simulink model "P2_B"  (R2024b)
settings: Solver=VariableStepAuto  StartTime=0.0  StopTime=10.0  RelTol=1e-3
values from neighbouring files (symbols this model uses):
  B = 0.3    [p13.m]    (also in p15.m; p16.m)
undefined symbols (not defined in the file or in its folder): s, X, Y
settings Model: Creator=sepeh  LastModifiedBy=sepeh

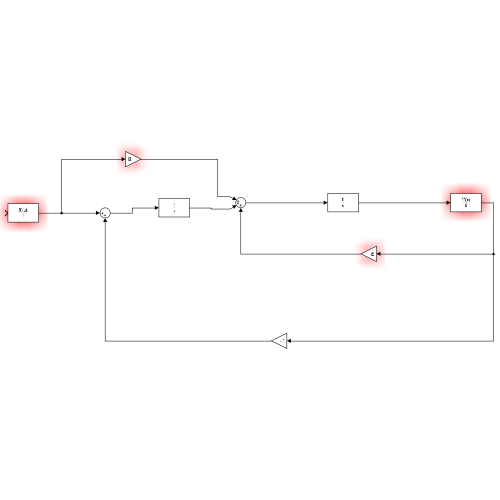
[thumbnail: Simulink's stored preview of the top-level diagram]
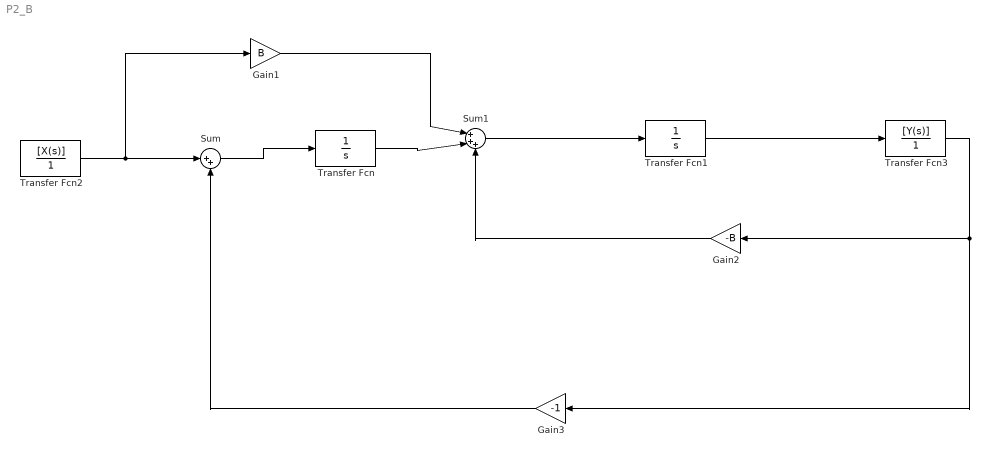
== system P2_B ==
  Gain1 : Gain  Gain=B
  Gain2 : Gain  Gain=-B
  Gain3 : Gain  Gain=-1
  Sum : Sum  Inputs=|++
  Sum1 : Sum  Inputs=|+++
  Transfer Fcn : TransferFcn  Denominator="[1  0]"
  Transfer Fcn1 : TransferFcn  Denominator="[1  0]"
  Transfer Fcn2 : TransferFcn  Numerator=[X(s)]  Denominator="[0  1]"
  Transfer Fcn3 : TransferFcn  Numerator=[Y(s)]  Denominator="[0  1]"
  wires:
  Transfer Fcn1/1 -> Transfer Fcn3/1
  Sum1/1 -> Transfer Fcn1/1
  Transfer Fcn3/1 -> Gain2/1, Gain3/1
  Gain2/1 -> Sum1/3
  Transfer Fcn/1 -> Sum1/2
  Transfer Fcn2/1 -> Gain1/1, Sum/1
  Sum/1 -> Transfer Fcn/1
  Gain1/1 -> Sum1/1
  Gain3/1 -> Sum/2
